simulink model "hdlcoder_byte2tuple_eml"  (R2026a)
settings: Solver=FixedStepDiscrete  StopTime=10  FixedStep=1
settings Model: Creator=The MathWorks, Inc.  LastModifiedBy=The MathWorks, Inc.
settings OptimizationCC: ConditionallyExecuteInputs=off  InitFltsAndDblsToZero=on
settings DebuggingCC: AlgebraicLoopMsg=error  UnderspecifiedInitializationDetection=Classic  SingleTaskRateTransMsg=error
settings HardwareCC: ProdHWDeviceType=ASIC/FPGA->ASIC/FPGA  ProdEqTarget=off
settings GRTTargetCC: CombineOutputUpdateFcns=off  GRTInterface=on

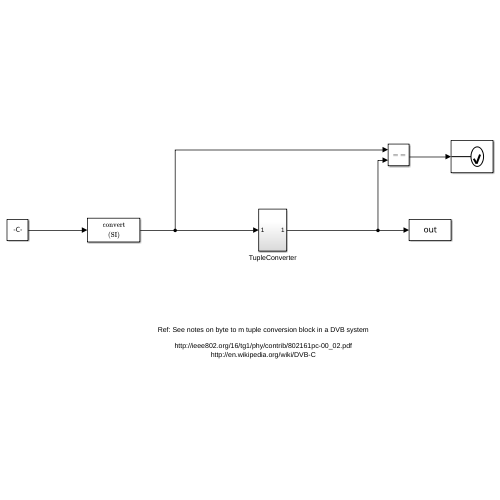
[thumbnail: Simulink's stored preview of the top-level diagram]
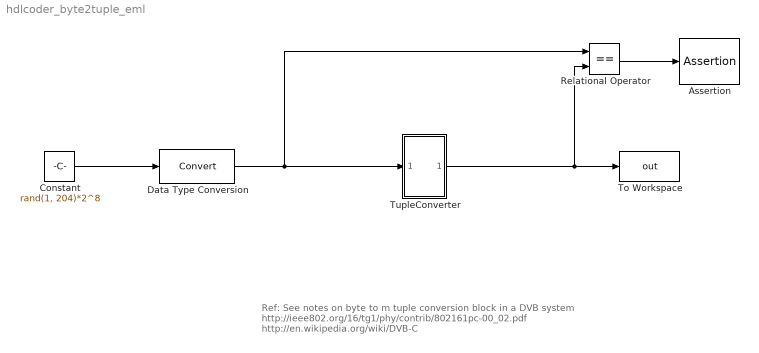
== system hdlcoder_byte2tuple_eml ==
  note: Ref: See notes on byte to m tuple conversion block in a DVB system
      |
      | http://ieee802.org/16/tg1/phy/contrib/802161pc-00_02.pdf
      | http://en.wikipedia.org/wiki/DVB-C
  Assertion : Assertion
  Constant : Constant  Value=rand(1, 204)*2^8  SampleTime=1
  Data Type Conversion : DataTypeConversion  ConvertRealWorld=Stored Integer (SI)  SaturateOnIntegerOverflow=off  RndMeth=Floor
  Relational Operator : RelationalOperator  Operator===  OutDataTypeStr=boolean  InputSameDT=off
  To Workspace : ToWorkspace  VariableName=out  SampleTime=-1
  TupleConverter : Subsystem
  wires:
  Constant/1 -> Data Type Conversion/1
  Data Type Conversion/1 -> Relational Operator/1, TupleConverter/1(In1)
  TupleConverter/1(Out1) -> Relational Operator/2, To Workspace/1
  Relational Operator/1 -> Assertion/1

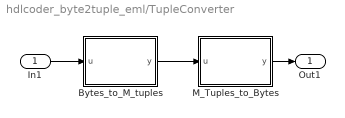
== system hdlcoder_byte2tuple_eml/TupleConverter ==
  In1 : Inport
  Bytes_to_M_tuples : MATLAB Function  TreatAsAtomicUnit=on
  M_Tuples_to_Bytes : MATLAB Function  TreatAsAtomicUnit=on
  Out1 : Outport
  wires:
  Bytes_to_M_tuples/1(y) -> M_Tuples_to_Bytes/1(u)
  In1/1 -> Bytes_to_M_tuples/1(u)
  M_Tuples_to_Bytes/1(y) -> Out1/1

== matlab function hdlcoder_byte2tuple_eml/TupleConverter/M_Tuples_to_Bytes ==
  data: u input fixdt(0,6,0) size=272; y output uint8
function y = fcn(u)
% convert M tuples to Bytes

% This particular example uses bitwise slice and concat operations 
% to convert a frame of words 272x6 (6bit tuples) to 204x8 (bytes).

% The following algorithm works on 4 tuples at a time 

inpFrameLen = length(u);
symbolWL    = 6; % Number of bits per M-ary symbol (word length), M = 64
outFrameLen = symbolWL*inpFrameLen / 8;

% Initialize output index counter, dimensions, and data type
% ----------------------------------------------------------
out_idx = int32(1);
% Use the FI equivalent to uint8 (for bitwise ops below)
yt = fi(zeros(outFrameLen,1), 0, 8, 0);

% Do the byte to m-tuple conversion
% ---------------------------------
for inp_idx = int32(1:4:inpFrameLen)
    % Get next four (ufix6) input words
    i1 = u(inp_idx);
    i2 = u(inp_idx+1);
    i3 = u(inp_idx+2);
    i4 = u(inp_idx+3);
    
    % Form next three (uint8) output words
    % starting with the MSB of the first word
    yt(out_idx)   = bitconcat(i1,                    bitsliceget(i2, 6, 5));
    yt(out_idx+1) = bitconcat(bitsliceget(i2, 4, 1), bitsliceget(i3, 6, 3));
    yt(out_idx+2) = bitconcat(bitsliceget(i3, 2, 1), i4);
    
    % Increment out_idx for next time through loop
    out_idx = out_idx + 3;
end

y = uint8(yt);

== matlab function hdlcoder_byte2tuple_eml/TupleConverter/Bytes_to_M_tuples ==
  data: u input uint8 size=204; y output fixdt(0,6,0)
function y = fcn(u)
% convert Bytes to M tuples

% This particular example uses bitwise slice and concat operations 
% to convert a frame of words 204x8 (bytes) to 272x6 (6bit tuples).

% The following algorithm works on 3 bytes at a time 

symbolWL    = 6; % Number of bits per M-ary symbol (word length), M = 64
inpFrameLen = length(u);
outFrameLen = 8*inpFrameLen / symbolWL;

% Initialize output index counter, dimensions, and data type
% ----------------------------------------------------------
out_idx = int32(1);
y       = fi(zeros(outFrameLen,1),0,6,0);

% Do the byte to m-tuple conversion
% ---------------------------------
nt = numerictype(0, 8, 0); % FI equivalent to uint8 (for bitwise ops below)
for inp_idx = int32(1:3:inpFrameLen)
    % Get next three (uint8) input words
    a = fi(u(inp_idx),   nt);
    b = fi(u(inp_idx+1), nt);
    c = fi(u(inp_idx+2), nt);
    
    % Form next four (ufix6) output words
    % starting with the MSB of the first word
    y(out_idx)   = bitsliceget(a, 8, 3);
    y(out_idx+1) = bitconcat(bitsliceget(a, 2, 1), bitsliceget(b, 8, 5));
    y(out_idx+2) = bitconcat(bitsliceget(b, 4, 1), bitsliceget(c, 8, 7));
    y(out_idx+3) = bitsliceget(c, 6, 1);
    
    % Increment out_idx for next time through loop
    out_idx = out_idx + 4;
end
